simulink model "ECU"  (R2025b)
settings: Solver=VariableStepAuto  StartTime=0.0  StopTime=inf  FixedStep=ts  RelTol=1e-3  EnableMultiTasking=on
model workspace (MAT data in the model file):
  AFRStoich = Simulink.Parameter
  AFRStoich.Value = 14.6
  AFRStoich.Complexity = 'real'
  AFRStoich.Dimensions = [1 1]
  AFRStoich.DataType = 'double'
  AirIdealGasCnst = Simulink.Parameter
  AirIdealGasCnst.Value = 287
  AirIdealGasCnst.Complexity = 'real'
  AirIdealGasCnst.Dimensions = [1 1]
  AirIdealGasCnst.DataType = 'double'
  AirMassFlowCorrEngLdBpt = Simulink.Parameter
  AirMassFlowCorrEngLdBpt.Value = [0.223381333333 0.285105122807 0.346828912281 0.408552701754 0.470276491228 0.532000280702 0.593724070175 0.655447859649 0.717171649123 0.778895438596 0.84061922807 0.902343017544 0.964066807018 1.02579059649 1.08751438596 1.14923817544 1.21096196491 1.27268575439 1.33440954386 1.39613333333]
  AirMassFlowCorrEngLdBpt.Complexity = 'real'
  AirMassFlowCorrEngLdBpt.Dimensions = [1 20]
  AirMassFlowCorrEngLdBpt.DataType = 'double'
  AirMassFlwCorrEngSpdBpt = Simulink.Parameter
  AirMassFlwCorrEngSpdBpt.Value = [750 973.6842 1197.3684 1421.0526 1644.7368 1868.4211 2092.1053 2315.7895 2539.4737 2763.1579 2986.8421 3210.5263 3434.2105 3657.8947 3881.5789 4105.2632 4328.9474 4552.6316 4776.3158 5000]
  AirMassFlwCorrEngSpdBpt.Complexity = 'real'
  AirMassFlwCorrEngSpdBpt.Dimensions = [1 20]
  AirMassFlwCorrEngSpdBpt.DataType = 'double'
  AirMassFlwCorrTbl = Simulink.Parameter
  AirMassFlwCorrTbl.Value = [1.02156051768 1.00597426471 0.989411677851 1.0033499089 0.984591437857 0.988509040623 1.0326198627 1.02765527362 1.0134784519 0.998280021213 0.981755128787 0.967218261288 ... (400 elements, 20x20)]
  AirMassFlwCorrTbl.Complexity = 'real'
  AirMassFlwCorrTbl.Dimensions = [20 20]
  AirMassFlwCorrTbl.DataType = 'double'
  CatLightOffTime = Simulink.Parameter
  CatLightOffTime.Value = 0
  CatLightOffTime.Complexity = 'real'
  CatLightOffTime.Dimensions = [1 1]
  CatLightOffTime.DataType = 'double'
  Cps = Simulink.Parameter
  Cps.Value = 2
  Cps.Complexity = 'real'
  Cps.Dimensions = [1 1]
  Cps.DataType = 'double'
  CylTrpdMassCorr = Simulink.Parameter
  CylTrpdMassCorr.Value = [0.839360054391 0.833393271885 0.82629554201 0.818442814437 0.811524387436 0.809164184856 0.814606352881 0.826887956871 0.842304598924 0.856886829014 0.869487025783 0.880530414174 ... (400 elements, 20x20)]
  CylTrpdMassCorr.Complexity = 'real'
  CylTrpdMassCorr.Dimensions = [20 20]
  CylTrpdMassCorr.DataType = 'double'
  DesiredIdleSpeed = Simulink.Parameter
  DesiredIdleSpeed.Value = 750
  DesiredIdleSpeed.Complexity = 'real'
  DesiredIdleSpeed.Dimensions = [1 1]
  DesiredIdleSpeed.DataType = 'double'
  ECP_Table = Simulink.Parameter
  ECP_Table.Value = [0 0 7.19012817097 15.3709456879 19.1470470057 19.0854874367 13.5819971805 0 0 0 0 0 ... (240 elements, 16x15)]
  ECP_Table.Complexity = 'real'
  ECP_Table.Dimensions = [16 15]
  ECP_Table.DataType = 'double'
  EngSpdBpt = Simulink.Parameter
  EngSpdBpt.Value = [750 973.6842 1197.3684 1421.0526 1644.7368 1868.4211 2092.1053 2315.7895 2539.4737 2763.1579 2986.8421 3210.5263 3434.2105 3657.8947 3881.5789 4105.2632 4328.9474 4552.6316 4776.3158 5000]
  EngSpdBpt.Complexity = 'real'
  EngSpdBpt.Dimensions = [1 20]
  EngSpdBpt.DataType = 'double'
  EngStopStartEnable = Simulink.Parameter
  EngStopStartEnable.Value = 1
  EngStopStartEnable.Complexity = 'real'
  EngStopStartEnable.Dimensions = [1 1]
  EngStopStartEnable.DataType = 'boolean'
  EngStopTime = Simulink.Parameter
  EngStopTime.Value = 5
  EngStopTime.Complexity = 'real'
  EngStopTime.Dimensions = [1 1]
  EngStopTime.DataType = 'auto'
  ExhCamPhaseBpt = Simulink.Parameter
  ExhCamPhaseBpt.Value = [0 2.6316 5.2632 7.8947 10.5263 13.1579 15.7895 18.4211 21.0526 23.6842 26.3158 28.9474 31.5789 34.2105 36.8421 39.4737 42.1053 44.7368 47.3684 50]
  ExhCamPhaseBpt.Complexity = 'real'
  ExhCamPhaseBpt.Dimensions = [1 20]
  ExhCamPhaseBpt.DataType = 'double'
  ExhGasTmpLdBpt = Simulink.Parameter
  ExhGasTmpLdBpt.Value = [0.2 0.275 0.35 0.425 0.5 0.575 0.65 0.725 0.8 0.875 0.95 1.025 1.1 1.175 1.25]
  ExhGasTmpLdBpt.Complexity = 'real'
  ExhGasTmpLdBpt.Dimensions = [1 15]
  ExhGasTmpLdBpt.DataType = 'double'
  ExhGasTmpSpdBpt = Simulink.Parameter
  ExhGasTmpSpdBpt.Value = [750 1053.57142857 1357.14285714 1660.71428571 1964.28571429 2267.85714286 2571.42857143 2875 3178.57142857 3482.14285714 3785.71428571 4089.28571429 4392.85714286 4696.42857143 5000]
  ExhGasTmpSpdBpt.Complexity = 'real'
  ExhGasTmpSpdBpt.Dimensions = [1 15]
  ExhGasTmpSpdBpt.DataType = 'double'
  ExhGasTmpTbl = Simulink.Parameter
  ExhGasTmpTbl.Value = [739.936218766 750.584766028 772.770773797 791.235245621 803.106549716 885.862998064 920.498479307 920.498479307 920.498479307 920.498479307 920.498479307 920.498479307 ... (225 elements, 15x15)]
  ExhGasTmpTbl.Complexity = 'real'
  ExhGasTmpTbl.Dimensions = [15 15]
  ExhGasTmpTbl.DataType = 'double'
  FricTrqTbl = Simulink.Parameter
  FricTrqTbl.Value = [4.16  4.8  5.44  6.05  6.64  7.23  7.81  8.39  8.97  9.54  10.1  10.7  11.3  11.9  12.5; 4.42  5.07  5.69  6.29  6.89  7.49  8.09  8.69  9.28  9.86  10.4  11  11.6  12.2  12.8; 4.69  5.36  5.98  6.58  7.18  7.79  8.41  9.02  9.62  10.2  10.8  11.4  11.9  12.5  13.1; 4.88  5.59  6.25  6.87  7.48  8.09  8.71  9.32  9.92  10.5  11.1  11.7  12.3  12.9  13.4; 4.94  5.74  6.45  7.12  7.75  8.37  8.99  9.59  10.2  10.8  11.4  11.9  12.6  13.2  13.8; 4.93  5.76  6.56  7.29  7.97  8.62  9.23  9.83  10.4  11  11.6  12.2  12.8  13.4  14.1; 4.85  5.67  6.57  7.37  8.11  8.8  9.43  10  10.6  11.2  11.8  12.4  13  13.7  14.3; 4.74  5.57  6.46  7.34  8.14  8.88  9.55  10.2  10.8  11.4  12  12.6  13.2  13.8  14.4; 4.63  5.42  6.27  7.19  8.05  8.83  9.55  10.2  10.9  11.5  12.1  12.7  13.3  14  14.6; 4.52  5.29  6.11  6.98  7.84  8.65  9.4  10.1  10.8  11.5  12.1  12.8  13.4  14.1  14.6; 4.42  5.18  5.97  6.79  7.6  8.39  9.15  9.88  10.6  11.3  12.1  12.8  13.5  14.1  14.7; 4.34  5.09  5.86  6.64  7.42  8.17  8.88  9.6  10.3  11.1  11.9  12.7  13.4  14.1  14.7; 4.27  5.01  5.76  6.52  7.28  8.03  8.74  9.39  10.1  10.8  11.6  12.4  13.2  14  14.7; 4.21  4.94  5.67  6.42  7.16  7.89  8.59  9.25  9.93  10.7  11.5  12.3  13.1  13.8  14.6; 4.15  4.87  5.6  6.33  7.06  7.77  8.47  9.14  9.84  10.6  11.3  12.1  12.9  13.7  14.4]
  FricTrqTbl.Complexity = 'real'
  FricTrqTbl.Dimensions = [15 15]
  FricTrqTbl.DataType = 'double'
  ICP_Table = Simulink.Parameter
  ICP_Table.Value = [0 0 1 1.09273642197 2.29409401139 3.54274371837 0.947749647567 0 0 0 0 0 ... (240 elements, 16x15)]
  ICP_Table.Complexity = 'real'
  ICP_Table.Dimensions = [16 15]
  ICP_Table.DataType = 'double'
  InjSlp = Simulink.Parameter
  InjSlp.Value = 6.45161290323
  InjSlp.Complexity = 'real'
  InjSlp.Dimensions = [1 1]
  InjSlp.DataType = 'double'
  InrTrqEngSpdBpt = Simulink.Parameter
  InrTrqEngSpdBpt.Value = [750 1053.5714 1357.1429 1660.7143 1964.2857 2267.8571 2571.4286 2875 3178.5714 3482.1429 3785.7143 4089.2857 4392.8571 4696.4286 5000]
  InrTrqEngSpdBpt.Complexity = 'real'
  InrTrqEngSpdBpt.Dimensions = [1 15]
  InrTrqEngSpdBpt.DataType = 'double'
  InrTrqLdBpt = Simulink.Parameter
  InrTrqLdBpt.Value = [0.2 0.28571 0.37143 0.45714 0.54286 0.62857 0.71429 0.8 0.88571 0.97143 1.0571 1.1429 1.2286 1.3143 1.4]
  InrTrqLdBpt.Complexity = 'real'
  InrTrqLdBpt.Dimensions = [1 15]
  InrTrqLdBpt.DataType = 'double'
  InrTrqTbl = Simulink.Parameter
  InrTrqTbl.Value = [25.8508 37.8267 50.6081 62.6825 74.6026 88.9064 81.9508 76.6399 82.9886 85.0042 88.9209 92.7645 ... (225 elements, 15x15)]
  InrTrqTbl.Complexity = 'real'
  InrTrqTbl.Dimensions = [15 15]
  InrTrqTbl.DataType = 'double'
  IntkCamPhaseBpt = Simulink.Parameter
  IntkCamPhaseBpt.Value = [0 2.6316 5.2632 7.8947 10.5263 13.1579 15.7895 18.4211 21.0526 23.6842 26.3158 28.9474 31.5789 34.2105 36.8421 39.4737 42.1053 44.7368 47.3684 50]
  IntkCamPhaseBpt.Complexity = 'real'
  IntkCamPhaseBpt.Dimensions = [1 20]
  IntkCamPhaseBpt.DataType = 'double'
  IntkMassFlw = Simulink.Parameter
  IntkMassFlw.Value = [0 0 0 0 0 0 0 0 0 0 0 0 ... (400 elements, 20x20)]
  IntkMassFlw.Complexity = 'real'
  IntkMassFlw.Dimensions = [20 20]
  IntkMassFlw.DataType = 'double'
  IntkVlvClsdCylVol = Simulink.Parameter
  IntkVlvClsdCylVol.Value = [0.37716 0.38164 0.38611 0.39033 0.39428 0.39795 0.40132 0.40441 0.40719 0.40967 0.41184 0.41372 0.41529 0.41656 0.41755 0.41825 0.41867 0.41884 0.41874 0.41865]
  IntkVlvClsdCylVol.Complexity = 'real'
  IntkVlvClsdCylVol.Dimensions = [1 20]
  IntkVlvClsdCylVol.DataType = 'double'
  LAM_Table = Simulink.Parameter
  LAM_Table.Value = [1  1  1  1  1  1  1  1  1  1  1  1  1  1  1; 1  1  1  1  1  1  1  1  1  1  1  1  1  1  1; 1  1  1  1  1  1  1  1  1  1  1  1  1  1  1; 1  1  1  1  1  1  1  1  1  1  1  1  1  1  1; 1  1  1  1  1  1  1  1  1  1  1  1  1  1  1; 1  1  1  1  1  1  1  1  1  1  1  1  1  1  1; 1  1  1  1  1  1  1  1  1  1  1  1  1  1  1; 1  1  1  1  1  1  1  1  1  1  1  1  1  1  1; 1  1  1  1  1  1  1  1  1  1  1  1  1  1  1; 1  1  1  1  1  1  1  1  1  1  1  1  1  1  1; 1  1  1  1  1  1  1  1  1  1  1  1  1  1  0.978833376279; 1  1  1  1  1  0.994115442909  1  0.972947102204  0.980523305065  0.999379925377  1  0.999606769395  0.999730304812  0.995941175028  0.966904774685; 1  1  1  0.94651624294  1  0.952506105741  0.994491417815  0.906466250495  0.924122061249  0.974767007025  0.985748891861  0.982416523617  0.992900047913  0.942109771144  0.941787575943; 1  1  1  0.942  0.937279637266  0.910896768573  0.929830385386  0.839985398785  0.854904769548  0.889462296842  0.92380217143  0.919912974116  0.958707785886  0.945711085936  0.914402970615; 1  1  1  0.942  0.902  0.869287431405  0.865169352957  0.81  0.824  0.812  0.837314196571  0.85940898562  0.888506841156  0.882667105929  0.87548189152; 1  1  1  0.942  0.902  0.846  0.824  0.81  0.824  0.812  0.826  0.818  0.815209011399  0.813810193086  0.836]
  LAM_Table.Complexity = 'real'
  LAM_Table.Dimensions = [16 15]
  LAM_Table.DataType = 'double'
  LOAD_Table = Simulink.Parameter
  LOAD_Table.Value = [0 0.337451044653 0.414402108642 0.494486992817 0.575342588384 0.624156549101 0.624156549101 0.624156549101 0.624156549101 0.624156549101 0.624156549101 0.624156549101 ... (240 elements, 16x15)]
  LOAD_Table.Complexity = 'real'
  LOAD_Table.Dimensions = [16 15]
  LOAD_Table.DataType = 'double'
  LamEffLamBp = Simulink.Parameter
  LamEffLamBp.Value = [0.65 0.7 0.75 0.8 0.85 0.9 0.95 1 1.05 1.1]
  LamEffLamBp.Complexity = 'real'
  LamEffLamBp.Dimensions = [1 10]
  LamEffLamBp.DataType = 'double'
  LamEffTbl = Simulink.Parameter
  LamEffTbl.Value = [0.94128 0.95565 0.97001 0.98437 0.99008 1.0004 0.97527 0.9549 0.92612 0.89735]
  LamEffTbl.Complexity = 'real'
  LamEffTbl.Dimensions = [1 10]
  LamEffTbl.DataType = 'double'
  Load_bp = Simulink.Parameter
  Load_bp.Value = [0 0.2 0.275 0.35 0.425 0.5 0.575 0.65 0.725 0.8 0.875 0.95 1.025 1.1 1.175 1.25]
  Load_bp.Complexity = 'real'
  Load_bp.Dimensions = [1 16]
  Load_bp.DataType = 'double'
  NCyl = Simulink.Parameter
  NCyl.Value = 4
  NCyl.Complexity = 'real'
  NCyl.Dimensions = [1 1]
  NCyl.DataType = 'double'
  NrmlzdDenBpt = Simulink.Parameter
  NrmlzdDenBpt.Value = [0.3 0.38947 0.47895 0.56842 0.65789 0.74737 0.83684 0.92632 1.0158 1.1053 1.1947 1.2842 1.3737 1.4632 1.5526 1.6421 1.7316 1.8211 1.9105 2]
  NrmlzdDenBpt.Complexity = 'real'
  NrmlzdDenBpt.Dimensions = [1 20]
  NrmlzdDenBpt.DataType = 'double'
  Pstd = Simulink.Parameter
  Pstd.Value = 101325
  Pstd.Complexity = 'real'
  Pstd.Dimensions = [1 1]
  Pstd.DataType = 'double'
  PumpTrqTbl = Simulink.Parameter
  PumpTrqTbl.Value = [7.24  7.7  7.82  7.95  8.1  8.27  8.45  8.64  8.78  8.88  8.96  9.03  9.12  9.25  9.45; 5.67  6.03  6.37  6.67  6.92  7.14  7.33  7.5  7.67  7.84  8.01  8.19  8.38  8.58  8.8; 3.94  4.52  5  5.36  5.6  5.77  5.92  6.1  6.35  6.67  7.02  7.4  7.75  8.06  8.34; 2.59  3.14  3.57  3.86  4.05  4.21  4.43  4.76  5.21  5.75  6.32  6.85  7.3  7.65  7.92; 1.8  2.25  2.61  2.88  3.11  3.37  3.71  4.17  4.74  5.36  5.96  6.49  6.91  7.23  7.46; 1  1.36  1.77  2.15  2.51  2.88  3.31  3.8  4.37  4.98  5.57  6.11  6.57  6.94  7.25; 1  1  1  1.09  1.59  2.08  2.6  3.17  3.81  4.49  5.19  5.85  6.44  6.92  7.29; 1  1  1  1  1  1.62  2.32  3.05  3.83  4.64  5.44  6.19  6.82  7.31  7.65; 1  1  1  1  1  1.35  2.21  3.08  3.97  4.88  5.78  6.64  7.41  8.06  8.58; 1  1  1  1  1  1  1.77  2.67  3.58  4.55  5.6  6.73  7.91  9.07  10.1; 1  1  1  1  1  1  1.72  2.67  3.61  4.62  5.79  7.15  8.69  10.3  11.9; 1  1  1  1  1  1  1.74  2.88  3.96  5.08  6.36  7.86  9.57  11.4  13.2; 1  1  1  1  1  1  1.37  2.7  4.01  5.39  6.92  8.65  10.5  12.4  14.2; 1  1  1  1  1  1  1.28  2.66  4.14  5.72  7.43  9.28  11.2  13.1  14.8; 1  1  1  1  1  1  1.39  2.82  4.39  6.06  7.85  9.73  11.6  13.5  15.1]
  PumpTrqTbl.Complexity = 'real'
  PumpTrqTbl.Dimensions = [15 15]
  PumpTrqTbl.DataType = 'double'
  SA_Table = Simulink.Parameter
  SA_Table.Value = [9.05 9.05 16.4373253582 15.3405265461 13.6074880273 9.83352189562 3.89388784387 0 0 0 0 0 ... (240 elements, 16x15)]
  SA_Table.Complexity = 'real'
  SA_Table.Dimensions = [16 15]
  SA_Table.DataType = 'double'
  SAoptTbl = Simulink.Parameter
  SAoptTbl.Value = [35.3085 21.0105 10.3714 8.5076 7.1426 7.5656 -5.7766 -16.7061 -16.8345 -19.3546 -20.6085 -22.0872 ... (225 elements, 15x15)]
  SAoptTbl.Complexity = 'real'
  SAoptTbl.Dimensions = [15 15]
  SAoptTbl.DataType = 'double'
  Speed_bp = Simulink.Parameter
  Speed_bp.Value = [750 1053.57142857 1357.14285714 1660.71428571 1964.28571429 2267.85714286 2571.42857143 2875 3178.57142857 3482.14285714 3785.71428571 4089.28571429 4392.85714286 4696.42857143 5000]
  Speed_bp.Complexity = 'real'
  Speed_bp.Dimensions = [1 15]
  Speed_bp.DataType = 'double'
  SpkTrqEffDlt = Simulink.Parameter
  SpkTrqEffDlt.Value = [0 0.75 1.5 2.25 3 3.75 4.5 5.25 6 6.75 7.5 8.25 9 9.75 10.5 11.25 12 12.75 13.5 14.25 15 15.75 16.5 17.25 18 18.75 19.5 20.25 21 21.75 22.5 23.25 24 24.75 25.5 26.25 27 27.75 28.5 29.25 30 30.75 31.5 32.25 33 33.75 34.5 35.25 36 36.75 37.5 38.25 39 39.75 40.5 41.25 42 42.75 43.5 44.25 45 45.75 46.5 47.25 48]
  SpkTrqEffDlt.Complexity = 'real'
  SpkTrqEffDlt.Dimensions = [1 65]
  SpkTrqEffDlt.DataType = 'double'
  SpkTrqEffTbl = Simulink.Parameter
  SpkTrqEffTbl.Value = [1.0019 0.9988 0.9953 0.99173 0.98811 0.98441 0.98065 0.97682 0.97293 0.96897 0.96493 0.96083 0.95666 0.95242 0.94811 0.94373 0.93927 0.93475 0.93015 0.92548 0.92074 0.91592 0.91104 0.90608 0.90105 0.89594 0.89076 0.88551 0.88019 0.8748 0.86933 0.86379 0.85818 0.8525 0.84675 0.84093 0.83503 0.82907 0.82303 0.81693 0.81075 0.80451 0.79819 0.79181 0.78536 0.77884 0.77226 0.7656 0.75888 0.75209 0.74524 0.73832 0.73134 0.72429 0.71717 0.70999 0.70275 0.69682 0.68949 0.68303 0.67548 0.67037 0.66525 0.66014 0.65503]
  SpkTrqEffTbl.Complexity = 'real'
  SpkTrqEffTbl.Dimensions = [1 65]
  SpkTrqEffTbl.DataType = 'double'
  TAP2TPP_Table = Simulink.Parameter
  TAP2TPP_Table.Value = [0 100]
  TAP2TPP_Table.Complexity = 'real'
  TAP2TPP_Table.Dimensions = [1 2]
  TAP2TPP_Table.DataType = 'double'
  TAP2TPP_bp = Simulink.Parameter
  TAP2TPP_bp.Value = [0 100]
  TAP2TPP_bp.Complexity = 'real'
  TAP2TPP_bp.Dimensions = [1 2]
  TAP2TPP_bp.DataType = 'double'
  TAP_Table = Simulink.Parameter
  TAP_Table.Value = [0 0.788736979167 0.788736979167 1.02768195697 1.31310759821 1.71307811728 2.2936923368 2.83561197917 2.83561197917 2.83561197917 2.83561197917 2.83561197917 ... (240 elements, 16x15)]
  TAP_Table.Complexity = 'real'
  TAP_Table.Dimensions = [16 15]
  TAP_Table.DataType = 'double'
  Torque_bp = Simulink.Parameter
  Torque_bp.Value = [0 15 26.4285714286 37.8571428571 49.2857142857 60.7142857143 72.1428571429 83.5714285714 95 106.428571429 117.857142857 129.285714286 140.714285714 152.142857143 163.571428571 175]
  Torque_bp.Complexity = 'real'
  Torque_bp.Dimensions = [1 16]
  Torque_bp.DataType = 'double'
  TrpdMassFlwBpt = Simulink.Parameter
  TrpdMassFlwBpt.Value = [0 5.7895 11.5789 17.3684 23.1579 28.9474 34.7368 40.5263 46.3158 52.1053 57.8947 63.6842 69.4737 75.2632 81.0526 86.8421 92.6316 98.4211 104.2105 110]
  TrpdMassFlwBpt.Complexity = 'real'
  TrpdMassFlwBpt.Dimensions = [1 20]
  TrpdMassFlwBpt.DataType = 'double'
  TrqLdSpdTbl = Simulink.Parameter
  TrqLdSpdTbl.Value = [15.0012133443 26.4298333923 37.8556656512 49.2846782956 60.7113978793 72.3451969202 77.459652163 78.5324534074 78.5324534074 78.5324534074 78.5324534074 78.5324534074 ... (225 elements, 15x15)]
  TrqLdSpdTbl.Complexity = 'real'
  TrqLdSpdTbl.Dimensions = [15 15]
  TrqLdSpdTbl.DataType = 'double'
  TrqLdSpdTblLdBpt = Simulink.Parameter
  TrqLdSpdTblLdBpt.Value = [0.2 0.275 0.35 0.425 0.5 0.575 0.65 0.725 0.8 0.875 0.95 1.025 1.1 1.175 1.25]
  TrqLdSpdTblLdBpt.Complexity = 'real'
  TrqLdSpdTblLdBpt.Dimensions = [1 15]
  TrqLdSpdTblLdBpt.DataType = 'double'
  TrqLdSpdTblSpdBpt = Simulink.Parameter
  TrqLdSpdTblSpdBpt.Value = [750 1053.57142857 1357.14285714 1660.71428571 1964.28571429 2267.85714286 2571.42857143 2875 3178.57142857 3482.14285714 3785.71428571 4089.28571429 4392.85714286 4696.42857143 5000]
  TrqLdSpdTblSpdBpt.Complexity = 'real'
  TrqLdSpdTblSpdBpt.Dimensions = [1 15]
  TrqLdSpdTblSpdBpt.DataType = 'double'
  Ts = Simulink.Parameter
  Ts.Value = 0.01
  Ts.Complexity = 'real'
  Ts.Dimensions = [1 1]
  Ts.DataType = 'auto'
  Tstd = Simulink.Parameter
  Tstd.Value = 293.15
  Tstd.Complexity = 'real'
  Tstd.Dimensions = [1 1]
  Tstd.DataType = 'double'
  Vd = Simulink.Parameter
  Vd.Value = 0.0015
  Vd.Complexity = 'real'
  Vd.Dimensions = [1 1]
  Vd.DataType = 'double'
  VolEffEngSpdBpt = Simulink.Parameter
  VolEffEngSpdBpt.Value = [750 1053.57142857 1357.14285714 1660.71428571 1964.28571429 2267.85714286 2571.42857143 2875 3178.57142857 3482.14285714 3785.71428571 4089.28571429 4392.85714286 4696.42857143 5000]
  VolEffEngSpdBpt.Complexity = 'real'
  VolEffEngSpdBpt.Dimensions = [1 15]
  VolEffEngSpdBpt.DataType = 'double'
  VolEffMapBpt = Simulink.Parameter
  VolEffMapBpt.Value = [31 40.6428571429 50.2857142857 59.9285714286 69.5714285714 79.2142857143 88.8571428571 98.5 108.142857143 117.785714286 127.428571429 137.071428571 146.714285714 156.357142857 166]
  VolEffMapBpt.Complexity = 'real'
  VolEffMapBpt.Dimensions = [1 15]
  VolEffMapBpt.DataType = 'double'
  VolEffTbl = Simulink.Parameter
  VolEffTbl.Value = [0.64175366561 0.641419295169 0.640125365558 0.638690556197 0.644169906538 0.669178791311 0.731659452876 0.750078238889 0.750078238889 0.750078238889 0.750078238889 0.750078238889 ... (225 elements, 15x15)]
  VolEffTbl.Complexity = 'real'
  VolEffTbl.Dimensions = [15 15]
  VolEffTbl.DataType = 'double'
  WAP_Table = Simulink.Parameter
  WAP_Table.Value = [100 100 100 100 100 100 100 100 100 100 100 100 ... (240 elements, 16x15)]
  WAP_Table.Complexity = 'real'
  WAP_Table.Dimensions = [16 15]
  WAP_Table.DataType = 'double'
  f_egr_areapct_cmd = Simulink.Parameter
  f_egr_areapct_cmd.Value = [0 3.448 6.897 10.34 13.79 17.24 20.69 24.14 27.59 31.03 34.48 37.93 ... (600 elements, 30x20)]
  f_egr_areapct_cmd.Complexity = 'real'
  f_egr_areapct_cmd.Dimensions = [30 20]
  f_egr_areapct_cmd.DataType = 'double'
  f_egr_areapct_nrmlzdflow_bpt = Simulink.Parameter
  f_egr_areapct_nrmlzdflow_bpt.Value = [0 0.03448 0.06897 0.1034 0.1379 0.1724 0.2069 0.2414 0.2759 0.3103 0.3448 0.3793 0.4138 0.4483 0.4828 0.5172 0.5517 0.5862 0.6207 0.6552 0.6897 0.7241 0.7586 0.7931 0.8276 0.8621 0.8966 0.931 0.9655 1]
  f_egr_areapct_nrmlzdflow_bpt.Complexity = 'real'
  f_egr_areapct_nrmlzdflow_bpt.Dimensions = [1 30]
  f_egr_areapct_nrmlzdflow_bpt.DataType = 'double'
  f_egr_areapct_pr_bpt = Simulink.Parameter
  f_egr_areapct_pr_bpt.Value = [0.5; 0.5263; 0.5526; 0.5789; 0.6053; 0.6316; 0.6579; 0.6842; 0.7105; 0.7368; 0.7632; 0.7895; 0.8158; 0.8421; 0.8684; 0.8947; 0.9211; 0.9474; 0.9737; 1]
  f_egr_areapct_pr_bpt.Complexity = 'real'
  f_egr_areapct_pr_bpt.Dimensions = [20 1]
  f_egr_areapct_pr_bpt.DataType = 'double'
  f_egr_max_stdflow = Simulink.Parameter
  f_egr_max_stdflow.Value = [74.87 74.87 74.74 74.39 73.81 72.98 71.91 70.58 68.97 67.06 64.84 62.25 59.27 55.81 51.79 47.07 36.33 24.22 12.11 0]
  f_egr_max_stdflow.Complexity = 'real'
  f_egr_max_stdflow.Dimensions = [1 20]
  f_egr_max_stdflow.DataType = 'double'
  f_egr_stdflow = Simulink.Parameter
  f_egr_stdflow.Value = [0 3.743 7.487 11.23 14.97 18.72 22.46 26.2 29.95 33.69 37.43 41.18 ... (420 elements, 21x20)]
  f_egr_stdflow.Complexity = 'real'
  f_egr_stdflow.Dimensions = [21 20]
  f_egr_stdflow.DataType = 'double'
  f_egr_stdflow_egrap_bpt = Simulink.Parameter
  f_egr_stdflow_egrap_bpt.Value = [0; 5; 10; 15; 20; 25; 30; 35; 40; 45; 50; 55; 60; 65; 70; 75; 80; 85; 90; 95; 100]
  f_egr_stdflow_egrap_bpt.Complexity = 'real'
  f_egr_stdflow_egrap_bpt.Dimensions = [21 1]
  f_egr_stdflow_egrap_bpt.DataType = 'double'
  f_egr_stdflow_pr_bpt = Simulink.Parameter
  f_egr_stdflow_pr_bpt.Value = [0.5; 0.5263; 0.5526; 0.5789; 0.6053; 0.6316; 0.6579; 0.6842; 0.7105; 0.7368; 0.7632; 0.7895; 0.8158; 0.8421; 0.8684; 0.8947; 0.9211; 0.9474; 0.9737; 1]
  f_egr_stdflow_pr_bpt.Complexity = 'real'
  f_egr_stdflow_pr_bpt.Dimensions = [20 1]
  f_egr_stdflow_pr_bpt.DataType = 'double'
  f_egrpct_cmd = Simulink.Parameter
  f_egrpct_cmd.Value = [0  0  0  0  0  0  0  0  0  0  0  0  0  0  0; 0  0  0  0  0  0  0  0  0  0  0  0  0  0  0; 0  0  0  0  0  0  0  0  0  0  0  0  0  0  0; 0  0  0  0  0  0  0  0  0  0  0  0  0  0  0; 0  0  0  0  0  0  0  0  0  0  0  0  0  0  0; 0  0  0  0  0  0  0  0  0  0  0  0  0  0  0; 0  0  0  0  0  0  0  0  0  0  0  0  0  0  0; 0  0  0  0  0  0  0  0  0  0  0  0  0  0  0; 0  0  0  0  0  0  0  0  0  0  0  0  0  0  0; 0  0  0  0  0  0  0  0  0  0  0  0  0  0  0; 0  0  0  0  0  0  0  0  0  0  0  0  0  0  0; 0  0  0  0  0  0  0  0  0  0  0  0  0  0  0; 0  0  0  0  0  0  0  0  0  0  0  0  0  0  0; 0  0  0  0  0  0  0  0  0  0  0  0  0  0  0; 0  0  0  0  0  0  0  0  0  0  0  0  0  0  0; 0  0  0  0  0  0  0  0  0  0  0  0  0  0  0]
  f_egrpct_cmd.Complexity = 'real'
  f_egrpct_cmd.Dimensions = [16 15]
  f_egrpct_cmd.DataType = 'double'
  f_egrpct_ld_bpt = Simulink.Parameter
  f_egrpct_ld_bpt.Value = [0 0.2 0.275 0.35 0.425 0.5 0.575 0.65 0.725 0.8 0.875 0.95 1.025 1.1 1.175 1.25]
  f_egrpct_ld_bpt.Complexity = 'real'
  f_egrpct_ld_bpt.Dimensions = [1 16]
  f_egrpct_ld_bpt.DataType = 'double'
  f_egrpct_n_bpt = Simulink.Parameter
  f_egrpct_n_bpt.Value = [750 1054 1357 1661 1964 2268 2571 2875 3179 3482 3786 4089 4393 4696 5000]
  f_egrpct_n_bpt.Complexity = 'real'
  f_egrpct_n_bpt.Dimensions = [1 15]
  f_egrpct_n_bpt.DataType = 'double'
  f_fric_temp_bpt = Simulink.Parameter
  f_fric_temp_bpt.Value = [275 277 279 281 283 285 287 289 291 293 295 297 299 301 303 305 307 309 311 313 315 317 319 321 323 325 327 329 331 333 335 337 339 341 343 345 347 349 351 353 355 357 359 361 363 365]
  f_fric_temp_bpt.Complexity = 'real'
  f_fric_temp_bpt.Dimensions = [1 46]
  f_fric_temp_bpt.DataType = 'double'
  f_fric_temp_mod = Simulink.Parameter
  f_fric_temp_mod.Value = [3.986 2.616 2.132 1.946 1.839 1.747 1.672 1.608 1.551 1.499 1.462 1.415 1.363 1.314 1.275 1.248 1.223 1.195 1.173 1.15 1.134 1.113 1.097 1.082 1.065 1.051 1.039 1.025 1.01 1.001 0.9907 0.9802 0.9699 0.9595 0.9593 0.954 0.9415 0.9368 0.9285 0.923 0.9185 0.9093 0.9018 0.8989 0.8965 0.887]
  f_fric_temp_mod.Complexity = 'real'
  f_fric_temp_mod.Dimensions = [1 46]
  f_fric_temp_mod.DataType = 'double'
  f_intksys_stdflow_bpt = Simulink.Parameter
  f_intksys_stdflow_bpt.Value = [0 29.67 59.34 89.01 117.8 144.1 155.7 166 175.2 183.3 190.7 197 202.7 207.7 212.2 216.1 219.4 222.2 224.5 226.4]
  f_intksys_stdflow_bpt.Complexity = 'real'
  f_intksys_stdflow_bpt.Dimensions = [1 20]
  f_intksys_stdflow_bpt.DataType = 'double'
  f_intksys_stdflow_pr = Simulink.Parameter
  f_intksys_stdflow_pr.Value = [1 0.9789 0.9579 0.9368 0.9158 0.8947 0.8737 0.8526 0.8316 0.8105 0.7895 0.7684 0.7474 0.7263 0.7053 0.6842 0.6632 0.6421 0.6211 0.6]
  f_intksys_stdflow_pr.Complexity = 'real'
  f_intksys_stdflow_pr.Dimensions = [1 20]
  f_intksys_stdflow_pr.DataType = 'double'
  tau_egr = Simulink.Parameter
  tau_egr.Value = 0.2
  tau_egr.Complexity = 'real'
  tau_egr.Dimensions = [1 1]
  tau_egr.DataType = 'double'
undefined symbols (not defined in the file): ts
libraries: autolibengctrlr x1, autolibengctrlrcommon x1
settings Model: ModifiedByFormat=The MathWorks, Inc.  SimulationMode=accelerator  Creator=The MathWorks, Inc.  LastModifiedBy=The MathWorks, Inc.
settings SolverCC: AlgebraicLoopSolver=TrustRegion  MaxZcPerStep=1.0
settings DataIOCC: DSMLogging=off  ReturnWorkspaceOutputs=off
settings DebuggingCC: UnconnectedInputMsg=warning  UnconnectedOutputMsg=warning  UnconnectedLineMsg=warning  ArithmeticOperatorsInVariantConditions=warning
settings ModelReferenceCC: EnableRefExpFcnMdlSchedulingChecks=on
settings SFSimCC: SimUseLocalCustomCode=off  CustomCodeUndefinedFunction=UseInterfaceOnly
settings RTWCC: RTWUseLocalCustomCode=off  GPUComputeCapability=3.5  DLArmComputeVersion=19.05
settings CodeAppCC: StateflowObjectComments=on
settings GRTTargetCC: TargetLangStandard=C89/C90 (ANSI)
settings ConfigComp: CovMetricSettings=dsw  CovSaveCumulativeToWorkspaceVar=on  CovSaveSingleToWorkspaceVar=on  CovExternalEMLEnable=off

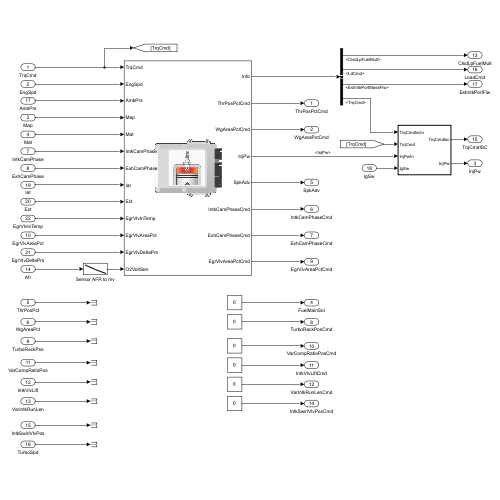
[thumbnail: Simulink's stored preview of the top-level diagram]
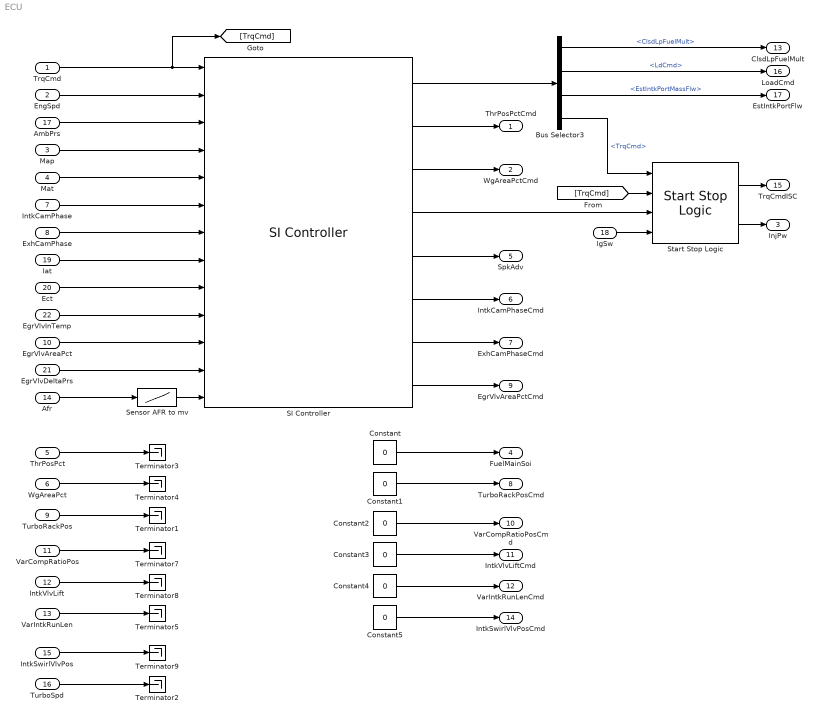
== system ECU ==
  TrqCmd : Inport
  EngSpd : Inport  Port=2
  Map : Inport  Port=3
  Mat : Inport  Port=4
  ThrPosPct : Inport  Port=5  Unit=%
  WgAreaPct : Inport  Port=6  Unit=%
  IntkCamPhase : Inport  Port=7
  ExhCamPhase : Inport  Port=8
  TurboRackPos : Inport  Port=9  Unit=1
  EgrVlvAreaPct : Inport  Port=10  Unit=%
  VarCompRatioPos : Inport  Port=11
  IntkVlvLift : Inport  Port=12
  VarIntkRunLen : Inport  Port=13
  Afr : Inport  Port=14  Unit=1
  IntkSwirlVlvPos : Inport  Port=15
  TurboSpd : Inport  Port=16  Unit=rpm
  AmbPrs : Inport  Port=17
  IgSw : Inport  Port=18
  Iat : Inport  Port=19  Unit=K
  Ect : Inport  Port=20  Unit=K
  EgrVlvDeltaPrs : Inport  Port=21  Unit=Pa
  EgrVlvInTemp : Inport  Port=22  Unit=K
  Bus Selector3 : BusSelector  OutputSignals=ClsdLpFuelMult,LdCmd,EstIntkPortMassFlw,TrqCmd
  Constant{,1..5} (6 alike) : Constant  Value=0  SampleTime=-1
  SI Controller : autolibengctrlr/SI Controller  AirEstOptionPopup=Dual Variable Cam Phasing  TrqEstOptionPopup=Torque Structure  f_lcmd=LOAD_Table  f_lcmd_tq_bpt=Torque_bp  f_lcmd_n_bpt=Speed_bp  f_tap=TAP_Table  f_tap_ld_bpt=Load_bp  f_tap_n_bpt=Speed_bp  f_tpp=TAP2TPP_Table  f_tpp_tap_bpt=TAP2TPP_bp  f_wap=WAP_Table  f_wap_ld_bpt=Load_bp  f_wap_n_bpt=Speed_bp  f_icp=ICP_Table  f_ecp=ECP_Table  f_cp_ld_bpt=Load_bp  f_cp_n_bpt=Speed_bp  f_egrpct_cmd=f_egrpct_cmd  f_egrpct_ld_bpt=f_egrpct_ld_bpt  f_egrpct_n_bpt=f_egrpct_n_bpt  f_egr_areapct_cmd=f_egr_areapct_cmd  f_egr_max_stdflow=f_egr_max_stdflow  f_egr_areapct_nrmlzdflow_bpt=f_egr_areapct_nrmlzdflow_bpt  f_egr_areapct_pr_bpt=f_egr_areapct_pr_bpt  LambdaCmdOvrd=off  Sinj=InjSlp  Nmin=1  afr_stoich=AFRStoich  f_lamcmd=LAM_Table  f_lamcmd_ld_bpt=Load_bp  f_lamcmd_n_bpt=Speed_bp  f_startup_lambda_delta=[0.5 0.3 0.2 0]  f_startup_lambda_delta_timecnst=[90 40 12 0]  f_startup_ect_bpt=[-40 0 20 50]  ClsdLpFuelEn=off  OpenLpDitherEn=off  LambdaDitherAmp=0.03  LambdaDitherFrq=0.75  ClsdLpFuelPGain=0.005  ClsdLpFuelIGain=0.05  ClsdLpFuelIntgLmt=0.2  O2ResetStoichVoltSen=2500  O2ResetMinVoltSen=0  O2ResetMaxVoltSen=5000  O2LearnUpdatePerSen=4  O2AmpMinVoltSen=250  O2ReadyVoltSen=1150  O2NotReadyVoltSen=1950  f_sa=SA_Table  f_sa_ld_bpt=Load_bp  f_sa_n_bpt=Speed_bp  N_idle=DesiredIdleSpeed  Trq_idlecmd_enable=1  Trq_idlecmd_max=50  Kp_idle=0.02  Ki_idle=0.01  EngRevLim=7000  CrankSpeed=150  ESSEnable=off  ESSExternalPortEnable=off  EngStopTime=5  CatLightOffTime=0  Ts=0.01  NCyl=NCyl  Cps=Cps  Vd=Vd  Rair=AirIdealGasCnst  Pstd=Pstd  Tstd=Tstd  f_nv=VolEffTbl  f_nv_prs_bpt=VolEffMapBpt  f_nv_n_bpt=VolEffEngSpdBpt  f_vivc=IntkVlvClsdCylVol  f_tm_corr_n_bpt=EngSpdBpt  f_vivc_icp_bpt=IntkCamPhaseBpt  f_tm_corr=CylTrpdMassCorr  f_tm_corr_nd_bpt=NrmlzdDenBpt  f_mdot_intk=IntkMassFlw  f_mdot_intk_ecp_bpt=ExhCamPhaseBpt  f_mdot_trpd_bpt=TrpdMassFlwBpt  f_mdot_air_corr=AirMassFlwCorrTbl  f_mdot_air_corr_ld_bpt=AirMassFlowCorrEngLdBpt  f_mdot_air_n_bpt=AirMassFlwCorrEngSpdBpt  tau_egr=tau_egr  f_intksys_stdflow_pr=f_intksys_stdflow_pr  f_intksys_stdflow_bpt=f_intksys_stdflow_bpt  f_egr_stdflow=f_egr_stdflow  f_egr_stdflow_pr_bpt=f_egr_stdflow_pr_bpt  f_egr_stdflow_egrap_bpt=f_egr_stdflow_egrap_bpt  f_tq_nl=TrqLdSpdTbl  f_tq_nl_l_bpt=TrqLdSpdTblLdBpt  f_tq_nl_n_bpt=TrqLdSpdTblSpdBpt  f_tq_inr=InrTrqTbl  f_tq_fric=FricTrqTbl  f_fric_temp_mod=f_fric_temp_mod  f_fric_temp_bpt=f_fric_temp_bpt  f_tq_pump=PumpTrqTbl  f_sa_opt=SAoptTbl  f_tq_inr_l_bpt=InrTrqLdBpt  f_tq_inr_n_bpt=InrTrqEngSpdBpt  f_m_sa=SpkTrqEffTbl  f_del_sa_bpt=SpkTrqEffDlt  f_m_lam=LamEffTbl  f_m_lam_bpt=LamEffLamBp  f_t_exh=ExhGasTmpTbl  f_t_exh_l_bpt=ExhGasTmpLdBpt  f_t_exh_n_bpt=ExhGasTmpSpdBpt
  Sensor AFR to mv : Lookup  InputValues="[14.4540   14.6000   14.7460]"  Table="[950   450    50]"  LookUpMeth=Interpolation-Use End Values  SaturateOnIntegerOverflow=off
  Start Stop Logic : autolibengctrlrcommon/Start Stop Logic  EngStopTime=EngStopTime  CatLightOffTime=CatLightOffTime  EngStopStartEnable=EngStopStartEnable  Ts=ts  aMode=1
  Terminator{1..5,7..9} (8 alike) : Terminator
  ThrPosPctCmd : Outport  VectorParamsAs1DForOutWhenUnconnected=off
  WgAreaPctCmd : Outport  Port=2  VectorParamsAs1DForOutWhenUnconnected=off
  InjPw : Outport  Port=3  Unit=ms  VectorParamsAs1DForOutWhenUnconnected=off
  FuelMainSoi : Outport  Port=4  Unit=deg  VectorParamsAs1DForOutWhenUnconnected=off
  SpkAdv : Outport  Port=5  VectorParamsAs1DForOutWhenUnconnected=off
  IntkCamPhaseCmd : Outport  Port=6  VectorParamsAs1DForOutWhenUnconnected=off
  ExhCamPhaseCmd : Outport  Port=7  VectorParamsAs1DForOutWhenUnconnected=off
  TurboRackPosCmd : Outport  Port=8  Unit=1  VectorParamsAs1DForOutWhenUnconnected=off
  EgrVlvAreaPctCmd : Outport  Port=9  Unit=%  VectorParamsAs1DForOutWhenUnconnected=off
  VarCompRatioPosCmd : Outport  Port=10  VectorParamsAs1DForOutWhenUnconnected=off
  IntkVlvLiftCmd : Outport  Port=11  VectorParamsAs1DForOutWhenUnconnected=off
  VarIntkRunLenCmd : Outport  Port=12  VectorParamsAs1DForOutWhenUnconnected=off
  ClsdLpFuelMult : Outport  Port=13  Unit=1  VectorParamsAs1DForOutWhenUnconnected=off
  IntkSwirlVlvPosCmd : Outport  Port=14  VectorParamsAs1DForOutWhenUnconnected=off
  TrqCmdISC : Outport  Port=15  Unit=N*m  VectorParamsAs1DForOutWhenUnconnected=off
  LoadCmd : Outport  Port=16  VectorParamsAs1DForOutWhenUnconnected=off
  EstIntkPortFlw : Outport  Port=17  VectorParamsAs1DForOutWhenUnconnected=off
  wires:
  SI Controller/2 -> ThrPosPctCmd/1
  EgrVlvInTemp/1 -> SI Controller/10
  Constant/1 -> FuelMainSoi/1
  Iat/1 -> SI Controller/8
  Start Stop Logic/1 -> TrqCmdISC/1
  IntkVlvLift/1 -> Terminator8/1
  Constant2/1 -> VarCompRatioPosCmd/1
  Ect/1 -> SI Controller/9
  EgrVlvAreaPct/1 -> SI Controller/11
  ThrPosPct/1 -> Terminator3/1
  Start Stop Logic/2 -> InjPw/1
  SI Controller/1 -> Bus Selector3/1
  Bus Selector3/2 -> LoadCmd/1  "<LdCmd>"
  IgSw/1 -> Start Stop Logic/4
  IntkSwirlVlvPos/1 -> Terminator9/1
  VarCompRatioPos/1 -> Terminator7/1
  Afr/1 -> Sensor AFR to mv/1
  Constant3/1 -> IntkVlvLiftCmd/1
  SI Controller/7 -> ExhCamPhaseCmd/1
  SI Controller/3 -> WgAreaPctCmd/1
  VarIntkRunLen/1 -> Terminator5/1
  SI Controller/5 -> SpkAdv/1
  Map/1 -> SI Controller/4
  EgrVlvDeltaPrs/1 -> SI Controller/12
  Constant4/1 -> VarIntkRunLenCmd/1
  WgAreaPct/1 -> Terminator4/1
  Mat/1 -> SI Controller/5
  AmbPrs/1 -> SI Controller/3
  TurboRackPos/1 -> Terminator1/1
  Constant5/1 -> IntkSwirlVlvPosCmd/1
  [TrqCmd] -> Start Stop Logic/2
  SI Controller/6 -> IntkCamPhaseCmd/1
  EngSpd/1 -> SI Controller/2
  Bus Selector3/4 -> Start Stop Logic/1  "<TrqCmd>"
  SI Controller/4 -> Start Stop Logic/3
  Constant1/1 -> TurboRackPosCmd/1
  ExhCamPhase/1 -> SI Controller/7
  TurboSpd/1 -> Terminator2/1
  TrqCmd/1 -> [TrqCmd], SI Controller/1
  Bus Selector3/3 -> EstIntkPortFlw/1  "<EstIntkPortMassFlw>"
  IntkCamPhase/1 -> SI Controller/6
  SI Controller/8 -> EgrVlvAreaPctCmd/1
  Sensor AFR to mv/1 -> SI Controller/13
  Bus Selector3/1 -> ClsdLpFuelMult/1  "<ClsdLpFuelMult>"
